simulink subsystem "theft_noise_model"  (R2025b)
settings: Solver=VariableStepAuto  StartTime=0.0  StopTime=10.0  RelTol=1e-3
settings Model: Creator=lenovo  LastModifiedBy=lenovo

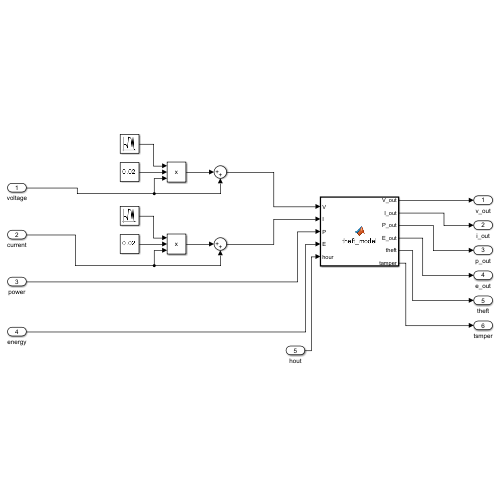
[thumbnail: Simulink's stored preview of the top-level diagram]
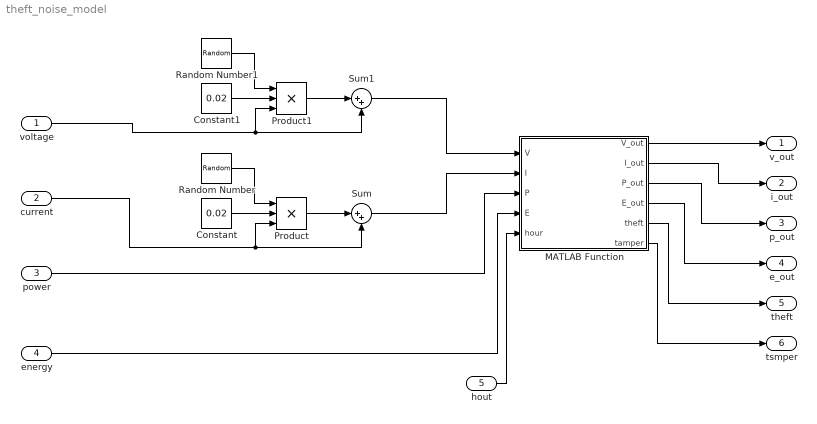
== system theft_noise_model ==
  voltage : Inport
  current : Inport  Port=2
  power : Inport  Port=3
  energy : Inport  Port=4
  hout : Inport  Port=5
  Constant : Constant  Value=0.02
  Constant1 : Constant  Value=0.02
  MATLAB Function : MATLAB Function  TreatAsAtomicUnit=on
  Product : Product  Inputs=3
  Product1 : Product  Inputs=3
  Random Number : RandomNumber  SampleTime=0.1
  Random Number1 : RandomNumber  SampleTime=0.1
  Sum : Sum  Inputs=|++
  Sum1 : Sum  Inputs=|++
  v_out : Outport
  i_out : Outport  Port=2
  p_out : Outport  Port=3
  e_out : Outport  Port=4
  theft : Outport  Port=5
  tsmper : Outport  Port=6
  wires:
  Constant/1 -> Product/2
  Random Number/1 -> Product/1
  current/1 -> Sum/2, Product/3
  Product/1 -> Sum/1
  Constant1/1 -> Product1/2
  Product1/1 -> Sum1/1
  Random Number1/1 -> Product1/1
  voltage/1 -> Sum1/2, Product1/3
  Sum1/1 -> MATLAB Function/1(V)
  Sum/1 -> MATLAB Function/2(I)
  power/1 -> MATLAB Function/3(P)
  energy/1 -> MATLAB Function/4(E)
  hout/1 -> MATLAB Function/5(hour)
  MATLAB Function/1(V_out) -> v_out/1
  MATLAB Function/2(I_out) -> i_out/1
  MATLAB Function/3(P_out) -> p_out/1
  MATLAB Function/4(E_out) -> e_out/1
  MATLAB Function/5(theft) -> theft/1
  MATLAB Function/6(tamper) -> tsmper/1

== matlab function theft_noise_model/MATLAB Function ==
  data: V input; V_out output; I input; P input; E input; hour input; I_out output; P_out output; E_out output; theft output; tamper output
function [V_out, I_out, P_out, E_out, theft, tamper] = theft_model(V, I, P, E, hour)

V_out = V;
I_out = I;
P_out = P;
E_out = E;

theft = 0;
tamper = 0;

r = rand;

% Type 1: Partial theft
if r < 0.1
    I_out = 0.6 * I;
    theft = 1;
end

% Type 2: Full bypass
if r >= 0.1 && r < 0.15
    I_out = 0;
    theft = 2;
end

% Type 3: Night theft
if (hour >= 22 || hour <= 5) && rand < 0.1
    I_out = 0.5 * I;
    theft = 3;
end

% Type 4: Data tampering
if rand < 0.05
    P_out = P + 200*randn;
    tamper = 1;
end

end
